simulink library "casper_library_delays"  (R2021a)
settings: Solver=ode45  StartTime=0.0  StopTime=10.0  RelTol=1e-3
libraries: xbsIndex_r4 x373, casper_library_misc x18, $bdroot x18, xbsReplacements_r4 x5, casper_library_multipliers x4, casper_library_downconverter x2
(part 1 of 5)
settings Model: Creator=mdexter  LastModifiedBy=jkocz
settings SolverCC: AlgebraicLoopSolver=TrustRegion
settings DataIOCC: LimitDataPoints=on  SaveFormat=Array  SignalLoggingSaveFormat=ModelDataLogs  ReturnWorkspaceOutputs=off
settings OptimizationCC: BlockReduction=off  BooleanDataType=off  ExpressionDepthLimit=2147483647  LifeSpan=inf
settings DebuggingCC: SaveWithParameterizedLinksMsg=none  UnderspecifiedInitializationDetection=Classic  MergeDetectMultiDrivingBlocksExec=none  SignalResolutionControl=TryResolveAllWithWarning  FcnCallInpInsideContextMsg=warning  AllowSymbolicDim=off  StateNameClashWarn=warning  SFUnexpectedBacktrackingDiag=warning  SFNoUnconditionalDefaultTransitionDiag=warning  SFExecutionAtInitializationDiag=none  SFMachineParentedDataDiag=warning  ArithmeticOperatorsInVariantConditions=warning
settings HardwareCC: ProdBitPerPointer=32  ProdBitPerSizeT=32  ProdBitPerPtrDiffT=32  ProdLargestAtomicFloat=None  ProdIntDivRoundTo=Undefined  ProdEndianess=Unspecified  ProdWordSize=32  ProdHWDeviceType=32-bit Generic  TargetUnknown=on
settings ModelReferenceCC: PropagateSignalLabelsOutOfModel=off
settings SFSimCC: SimUseLocalCustomCode=off  CustomCodeUndefinedFunction=UseInterfaceOnly
settings RTWCC: RTWUseLocalCustomCode=off
settings CodeAppCC: StateflowObjectComments=on
settings GRTTargetCC: TargetLangStandard=C89/C90 (ANSI)  CombineOutputUpdateFcns=off  GRTInterface=on
settings ConfigComp: CovMetricSettings=dw  CovSaveCumulativeToWorkspaceVar=on  CovSaveSingleToWorkspaceVar=on  CovExternalEMLEnable=off

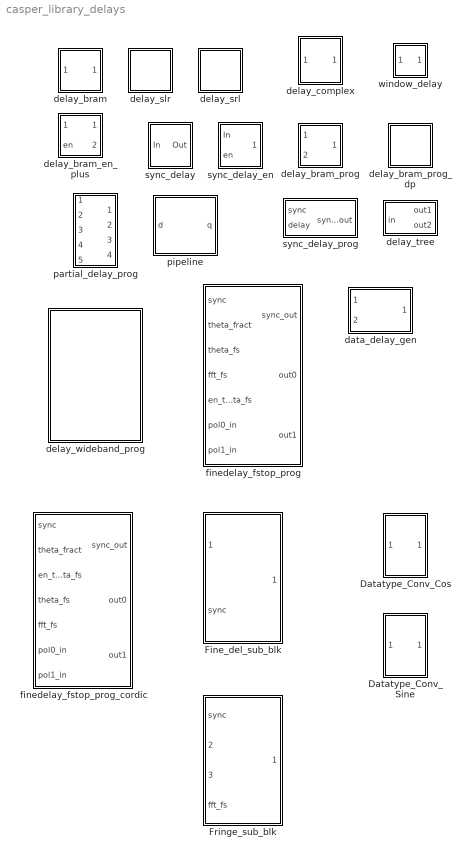
== system casper_library_delays ==
  Datatype_Conv_Cos : Subsystem  mask{theta_binary_bits=17, fft_bits=18}
      mask prompts: theta_binary_bits "Sine-Cos LUT Input binary point position"; fft_bits "FFT Input Bit Width"
  Datatype_Conv_Sine : Subsystem  mask{theta_binary_bits=17, fft_bits=18}
      mask prompts: theta_binary_bits "Sine-Cos LUT Input binary point position"; fft_bits "FFT Input Bit Width"
  Fine_del_sub_blk : Subsystem  mask{fft_len=1024, theta_bits=12, theta_binary_bits=9}
      mask prompts: fft_len "Number Of FFT Channels"; theta_bits "Sine-Cos LUT Input Bitwidth(Determines resolution of the phase)"; theta_binary_bits "Sine-Cos LUT Input binary point position"
      mask init:
      | low_limit = (2^theta_bits)*pi /8;
      | up_limit = (2^theta_bits)-((2^theta_bits)*pi /8);
  Fringe_sub_blk : Subsystem  mask{fft_len=1024, theta_bits=20, theta_binary_bits=17, fft_cycle_bits=17, sync_period=27}
      mask prompts: fft_len "Number Of FFT Channels"; theta_bits "Sine-Cos LUT Input Bitwidth (Determines the resolution of phase)"; theta_binary_bits "Sine-Cos LUT Input binary point position"; fft_cycle_bits "Maximum Number of FFT cycles  (Rate of change of Fringe ) = 2 ^ ?"; sync_period "Sync Period"
  data_delay_gen : Subsystem  mask(Delay_7){delaytype=sync_delay_prog, DelayLen=5, bram_latency=1, MaxDelay=1, use_dsp48=on}
      mask prompts: delaytype "delay type"; DelayLen "Delay by  [delay_bram, delay_slr, sync_delay, sync_delay_en, window_delay, pipeline]"; bram_latency "BRAM latency  [delay_bram]"; MaxDelay "Max Delay (2^?) [sync_delay_prog]"; use_dsp48 "Use DSP48 [delay_bram]"
      mask help: A combination of 7 different Delay blocks. Including delay_bram, delay_slr, sync_delay, sync_delay_en, sync_delay_prog, window_delay, pipeline.
      mask init:
      | config.source=str2func('delay_general');
      | config.name=delaytype;
      | config.toplevel=gcb;
      | xBlock(config, {delaytype, ...
      |                 {'Delaylen',DelayLen, ...
      |                 'MaxDelay', MaxDelay, ...
      |                 'use_dsp48', use_dsp48, ...
      |                 'bram_latency', bram_latency} }...
      |                 );
      settings: AttributesFormatString=Delay_7, %<delaytype>
      mask TypeOptions delaytype: delay_bram | delay_slr | sync_delay | sync_delay_en | sync_delay_prog | window_delay | pipeline
  delay_bram : Subsystem  mask(delay_bram){DelayLen=4, bram_latency=2, use_dsp48=off, async=off}
      mask prompts: DelayLen "Delay By:"; bram_latency "BRAM Latency"; use_dsp48 "Use DSP48"; async "asynchronous operation"
      mask help: A delay block that uses BRAM for its storage.
      mask init:
      | delay_bram_init(gcb, ...
      |     'DelayLen', DelayLen, ...
      |     'bram_latency', bram_latency, ...
      |     'use_dsp48', use_dsp48, ...
      |     'async', async);
      mask Help: eval('xlWeb(''http://casper.berkeley.edu/wiki/Delay_bram'')')
  delay_bram_en_plus : Subsystem  mask(delay_bram_en_plus){DelayLen=7, bram_latency=4}
      mask prompts: DelayLen "Enabled Delays:"; bram_latency "Extra (unenabled) delay for BRAM Latency"
      mask help:
      | A delay block that uses BRAM for its storage and only shifts when enabled.
      | However, BRAM latency cannot be enabled, so output appears <i>bram_latency</i>
      | clocks after an enable.
      mask init:
      | BitWidth = max(ceil(log2(DelayLen)), 2);
      mask Help: eval('xlWeb(''http://casper.berkeley.edu/wiki/Delay_bram_en_plus'')')
  delay_bram_prog : Subsystem  mask(delay_bram_prog){MaxDelay=7, bram_latency=4}
      mask prompts: MaxDelay "Max Delay (2^?):"; bram_latency "BRAM Latency"
      mask help:
      | A delay block that uses BRAM for its storage and has a run-time programmable
      | delay.  When delay is changed, some randomly determined samples will
      | be inserted/dropped from the buffered stream.
      mask Help: eval('xlWeb(''http://casper.berkeley.edu/wiki/Delay_bram_prog'')')
  delay_bram_prog_dp : Subsystem  mask(delay_bram_prog_dp){ram_bits=0, bram_latency=2, async=off}
      mask prompts: ram_bits "Max delay (2^?)"; bram_latency "BRAM latency"; async "asynchronous operation"
      mask init:
      | delay_bram_prog_dp_init(gcb, ...
      |     'ram_bits', ram_bits, ...
      |     'bram_latency', bram_latency, ...
      |     'async', async);
  delay_complex : Subsystem  mask(delay_complex){delay=6, n_bits=18, bin_pt=17, use_bram=1, bram_latency=3}
      mask prompts: delay "Delay Length"; n_bits "Sample Bit Width"; bin_pt "Binary Point"; use_bram "Use BRAM (0=no, 1=yes)"; bram_latency "BRAM Latency"
      mask help: A delay block that treats its input as complex, splits it into real and imaginary components, delays each component by a specified amount, and then re-joins them into a complex output. The underlying storage is user-selectable (either BRAM or SLR16 elements). The reason for this is wide (36 bit) delays make adjacent multipliers in multiplier-bram pairs unusable.
      mask init:
      | delay_complex_init(gcb, ...
      |     'delay', delay, ...
      |     'n_bits', n_bits, ...
      |     'bin_pt', bin_pt, ...
      |     'use_bram', use_bram, ...
      |     'bram_latency', bram_latency);
      settings: AttributesFormatString=|
      | depth = 6
      | delay_bram
      mask Help: eval('xlWeb(''http://casper.berkeley.edu/wiki/Delay_complex'')')
  delay_slr : Subsystem  mask(delay_slr){DelayLen=0, async=off}
      mask prompts: DelayLen "Delay by:"; async "asynchronous operation"
      mask help: A delay block that uses slices (SLR16s) for its storage.
      mask init:
      | delay_slr_init(gcb, ...
      |     'DelayLen', DelayLen, ...
      |     'async', async);
  delay_srl : Subsystem  mask(delay_srl){DelayLen=-1, async=off}
      mask prompts: DelayLen "Delay by:"; async "Asynchronous operation"
      mask help:
      | A delay block that uses slices (SRL16s) for its storage.
      |
      | It explicitly converts the first delay into a flip flop,
      | and lets XSG break up the remaining delays into a series
      | of SRL16+FF instances.
      |
      | This is advantageous because the setup time of an SRL is
      | longer than that of a flip flop.
      mask init:
      | delay_srl_init(gcb, ...
      |     'DelayLen', DelayLen, ...
      |     'async', async);
  delay_tree : Subsystem  mask(delay_tree){fanout=2, bfac=2}
      mask prompts: bfac "Branching factor"
      mask help: A tree of delays.
      mask init:
      | delay_tree_init(gcb, ...
      |     'fanout', fanout, ...
      |     'bfac', bfac);
      settings: AttributesFormatString=delay=2
  delay_wideband_prog : Subsystem  mask(delay_wideband_prog){max_delay=0, n_inputs_bits=2, bram_latency=2, bram_type=Dual Port, async=off}
      mask prompts: max_delay "Max Delay (Sample Clks)"; n_inputs_bits "Number of Simultaneous Inputs(2^?)"; bram_latency "BRAM Latency"; bram_type "Select type of BRAM"; async "asynchronous operation"
      mask init:
      | delay_wideband_prog_init(gcb,...
      |     'max_delay',max_delay,...
      |     'n_inputs_bits',n_inputs_bits,...
      |     'bram_latency',bram_latency,...
      |     'bram_type',bram_type, ...
      |     'async', async);
      mask TypeOptions bram_type: Single Port | Dual Port
  finedelay_fstop_prog : Subsystem  mask(finedelay_fstop_prog){n_input=2, fft_len=512, fft_bits=18, theta_bits=14, sine_cos_bits=18, fft_cycle_bits=12}
      mask prompts: n_input "Number of Simultaneous Inputs"; fft_len "Number Of FFT Channels"; fft_bits "FFT Input Bit Width"; theta_bits "Sine-Cos LUT Input Bitwidth (Determines the resolution of phase)"; sine_cos_bits "Sine-Cos LUT Output Data Width"; fft_cycle_bits "Maximum Number of FFT cycles  (Rate of change of Fringe ) = 2 ^ ?"
      mask init:
      | finedelay_fstop_prog_init(gcb,...
      |     'n_input',n_input,...
      |     'fft_len',fft_len,...
      |     'fft_bits',fft_bits,...
      |     'theta_bits',theta_bits,...
      |     'sine_cos_bits',sine_cos_bits,...
      |     'fft_cycle_bits',fft_cycle_bits);
  finedelay_fstop_prog_cordic : Subsystem  mask(finedelay_fstop_prog_cordic){n_input=2, fft_len=1024, fft_bits=18, theta_bits=20, theta_binary_bits=17, stages=9, fft_cycle_bits=17, sync_period=134217728}
      mask prompts: n_input "Number of Simultaneous Inputs"; fft_len "Number Of FFT Channels"; fft_bits "FFT Input Bit Width"; theta_bits "CORDIC Sine-Cos Input Bitwidth (Determines the resolution of phase)"; theta_binary_bits "CORDIC Sine-Cos Input Binary BitWidth"; stages "Number of Processing Elements of CORDIC block (integer value starting from 1)"; fft_cycle_bits "Maximum Number of FFT cycles  (Rate of change of Fringe ) = 2 ^ ?"; sync_period "Sync Period"
      mask init:
      | finedelay_fstop_prog_cordic_init(gcb,...
      |     'n_input',n_input,...
      |     'fft_len',fft_len,...
      |     'fft_bits',fft_bits,...
      |     'theta_bits',theta_bits,...
      |     'theta_binary_bits',theta_binary_bits,...
      |     'stages',stages,...
      |     'fft_cycle_bits',fft_cycle_bits,...
      |     'sync_period',sync_period);
  partial_delay_prog : Subsystem  mask(partial_delay){n_inputs=4, mux_latency=2}
      mask prompts: n_inputs "Number of Inputs (? >= 2)"; mux_latency "Mux Latency"
      mask help:
      | For a set of parallel inputs which represent consecutive time samples of the
      | same input signal, this block delays the stream by a dynamically selectable
      | number of samples between 0 and (n_inputs-1).
      mask init:
      | partial_delay_init(gcb, ...
      |     'n_inputs', n_inputs, ...
      |     'mux_latency', mux_latency);
      mask Help: eval('xlWeb(''http://casper.berkeley.edu/wiki/Partial_delay_prog'')')
  pipeline : Subsystem  mask(pipeline){csp_latency=3}
      mask prompts: csp_latency "Latency"
      mask help:
      | An explicitly laid-out delay line to avoid mapping to SRL16s
      | for use in pipelining to help achieve timing closure.
      mask init:
      | pipeline_init(gcb,'latency',csp_latency);
      settings: AttributesFormatString=Latency = %<latency>
      mask Display:
      | port_label('input', 1, 'd');
      | port_label('output', 1, 'q');
      | disp(['Z^-', num2str(csp_latency)]);
  sync_delay : Subsystem  mask(sync_delay){DelayLen=4}
      mask prompts: DelayLen "Delay Length:"
      mask help: Delay an infrequent boolean pulse by the specified number of clocks.
      mask init:
      | BitWidth = max(2, ceil(log2(DelayLen+1)));
      | UseCounter = 1;
      | if DelayLen == 0,
      | 	UseCounter = 0;
      | end
      mask Help: eval('xlWeb(''http://casper.berkeley.edu/wiki/Sync_delay'')')
      mask Display: fprintf('Z^-%d', DelayLen)
  sync_delay_en : Subsystem  mask(sync_delay_en){DelayLen=4}
      mask prompts: DelayLen "Delay Length:"
      mask help: Delay an infrequent boolean pulse by the specified number of enabled clocks.
      mask init:
      | BitWidth = max(2, ceil(log2(DelayLen+1)));
      | UseCounter = 1;
      | if DelayLen == 0,
      | 	UseCounter = 0;
      | end
      mask Help: eval('xlWeb(''http://casper.berkeley.edu/wiki/Sync_delay_en'')')
      mask Display:
      | fprintf('Z^-%d', DelayLen);
      | port_label('input',2,'en');
  sync_delay_prog : Subsystem  mask(sync_delay_prog){MaxDelay=4}
      mask prompts: MaxDelay "Max Delay (2^?):"
      mask help:
      | Delay an infrequent boolean pulse by  a run-time programmable number of enabled clocks.
      | If the input pulse repeats before the output pulse is generated, an internal counter
      | resets and that output pulse is never generated. When delay is changed, some randomly determined
      | samples will be inserted/dropped from the buffered stream.
      mask Help: eval('xlWeb(''http://casper.berkeley.edu/wiki/Sync_delay_prog'')')
  window_delay : Subsystem  mask{delay=10}
      mask prompts: delay "desired delay (>2)"
      mask Display: fprintf('Z^-%d', delay)

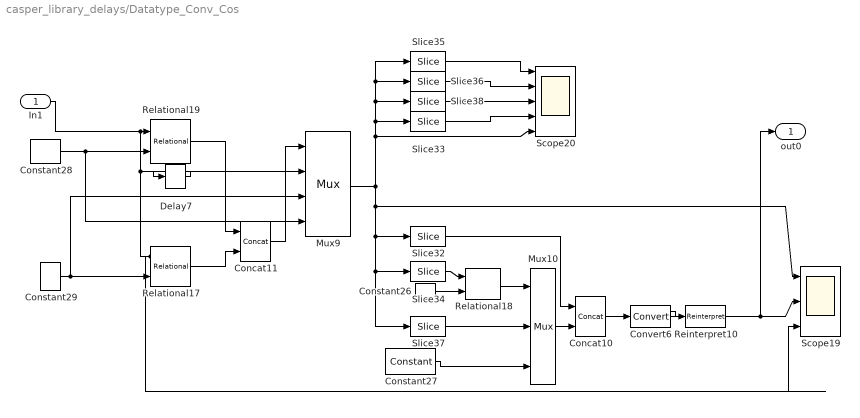
== system casper_library_delays/Datatype_Conv_Cos ==
  In1 : Inport
  Concat10 : xbsIndex_r4/Concat  num_inputs=2  dbl_ovrd=off  block_type=concat
      settings: block_version=10.1.3
  Concat11 : xbsIndex_r4/Concat  num_inputs=2  dbl_ovrd=off  block_type=concat
      settings: block_version=10.1.3
  Constant26 : xbsIndex_r4/Constant  const=1  gui_display_data_type=Fixed-point  arith_type=Unsigned  n_bits=3  bin_pt=0  preci_type=Single  exp_width=8  frac_width=24  explicit_period=off  period=1  equ=P=C  opselect=C  inp2=PCIN>>17  opr=+  inp1=P  carry=CIN  dbl_ovrd=off  block_type=constant
  Constant27 : xbsIndex_r4/Constant  const=2^(theta_binary_bits)-1  gui_display_data_type=Fixed-point  arith_type=Unsigned  n_bits=theta_binary_bits  bin_pt=0  preci_type=Single  exp_width=8  frac_width=24  explicit_period=off  period=1  equ=P=C  opselect=C  inp2=PCIN>>17  opr=+  inp1=P  carry=CIN  dbl_ovrd=off  block_type=constant
  Constant28 : xbsIndex_r4/Constant  const=1  gui_display_data_type=Fixed-point  arith_type=Signed (2's comp)  n_bits=20  bin_pt=17  preci_type=Single  exp_width=8  frac_width=24  explicit_period=off  period=1  equ=P=C  opselect=C  inp2=PCIN>>17  opr=+  inp1=P  carry=CIN  dbl_ovrd=off  block_type=constant
  Constant29 : xbsIndex_r4/Constant  const=-1  gui_display_data_type=Fixed-point  arith_type=Signed (2's comp)  n_bits=20  bin_pt=17  preci_type=Single  exp_width=8  frac_width=24  explicit_period=off  period=1  equ=P=C  opselect=C  inp2=PCIN>>17  opr=+  inp1=P  carry=CIN  dbl_ovrd=off  block_type=constant
  Convert6 : xbsIndex_r4/Convert  gui_display_data_type=Fixed-point  arith_type="Signed  (2's comp)"  n_bits=fft_bits  bin_pt=0  float_type=Single  exp_bits=8  fraction_bits=24  quantization=Truncate  overflow=Wrap  en=off  latency=0  pipeline=off  dbl_ovrd=off  block_type=convert
      settings: block_version=10.1.3
  Delay7 : xbsIndex_r4/Delay  rst=off  infoeditControl=Selection of Reset will increase slice count due to use of real FFs and instead of SRLs  en=off  latency=1  reg_retiming=off  dbl_ovrd=off  block_type=delay
  Mux10 : xbsIndex_r4/Mux  inputs=2  en=off  latency=0  precision=Full  arith_type=Unsigned  n_bits=16  bin_pt=14  quantization=Truncate  overflow=Wrap  dbl_ovrd=off  block_type=mux
  Mux9 : xbsIndex_r4/Mux  inputs=3  en=off  latency=0  precision=Full  arith_type=Unsigned  n_bits=16  bin_pt=14  quantization=Truncate  overflow=Wrap  dbl_ovrd=off  block_type=mux
  Reinterpret10 : xbsIndex_r4/Reinterpret  force_arith_type=off  arith_type=Unsigned  force_bin_pt=on  bin_pt=fft_bits-1  block_type=reinterpret
      settings: infoedit="Changes signal type without altering the binary representation.   You can changed the signal between signed and unsigned, and relocate the binary point.<P><P>Hardware notes: In hardware this block costs nothing.<P><P>Example:  Suppose the input is 6 bits wide, signed, with 2 fractional bits, and the output is forced to unsigned with 0 fractional bits.  Then an input of -2.0 (1110.00 in binary 2's complement) becomes an output of 56 (111000 in binary)."  block_version=10.1.3
  Relational17 : xbsIndex_r4/Relational  mode=a<b  op_type=Bool  en=off  latency=1  dbl_ovrd=off  block_type=relational
      settings: block_version=10.1.3
  Relational18 : xbsIndex_r4/Relational  mode=a=b  op_type=Bool  en=off  latency=0  dbl_ovrd=off  block_type=relational
      settings: block_version=10.1.3
  Relational19 : xbsIndex_r4/Relational  mode=a>b  op_type=Bool  en=off  latency=1  dbl_ovrd=off  block_type=relational
      settings: block_version=10.1.3
  Scope19 : Scope  NumInputPorts=3
  Scope20 : Scope  NumInputPorts=5
  Slice32 : xbsIndex_r4/Slice  nbits=1  boolean_output=off  mode=Upper Bit Location + Width  bit1=0  base1=MSB of Input  bit0=0  base0=LSB of Input  dbl_ovrd=off  block_type=slice
      settings: infoedit="Extracts a given range of bits from each input sample and presents it at the output.  The output type is ordinarily unsigned with binary point at zero, but can be Boolean when the slice is one bit wide.<P><P>Hardware notes: In hardware this block costs nothing."  block_version=10.1.3
  Slice33 : xbsIndex_r4/Slice  nbits=3  boolean_output=off  mode=Upper Bit Location + Width  bit1=0  base1=MSB of Input  bit0=0  base0=LSB of Input  dbl_ovrd=off  block_type=slice
      settings: infoedit="Extracts a given range of bits from each input sample and presents it at the output.  The output type is ordinarily unsigned with binary point at zero, but can be Boolean when the slice is one bit wide.<P><P>Hardware notes: In hardware this block costs nothing."  block_version=10.1.3
  Slice34 : xbsIndex_r4/Slice  nbits=3  boolean_output=off  mode=Upper Bit Location + Width  bit1=0  base1=MSB of Input  bit0=0  base0=LSB of Input  dbl_ovrd=off  block_type=slice
      settings: infoedit="Extracts a given range of bits from each input sample and presents it at the output.  The output type is ordinarily unsigned with binary point at zero, but can be Boolean when the slice is one bit wide.<P><P>Hardware notes: In hardware this block costs nothing."  block_version=10.1.3
  Slice35 : xbsIndex_r4/Slice  nbits=1  boolean_output=off  mode=Upper Bit Location + Width  bit1=0  base1=MSB of Input  bit0=0  base0=LSB of Input  dbl_ovrd=off  block_type=slice
      settings: infoedit="Extracts a given range of bits from each input sample and presents it at the output.  The output type is ordinarily unsigned with binary point at zero, but can be Boolean when the slice is one bit wide.<P><P>Hardware notes: In hardware this block costs nothing."  block_version=10.1.3
  Slice36 : xbsIndex_r4/Slice  nbits=1  boolean_output=off  mode=Upper Bit Location + Width  bit1=-1  base1=MSB of Input  bit0=0  base0=LSB of Input  dbl_ovrd=off  block_type=slice
      settings: infoedit="Extracts a given range of bits from each input sample and presents it at the output.  The output type is ordinarily unsigned with binary point at zero, but can be Boolean when the slice is one bit wide.<P><P>Hardware notes: In hardware this block costs nothing."  block_version=10.1.3
  Slice37 : xbsIndex_r4/Slice  nbits=theta_binary_bits  boolean_output=off  mode=Lower Bit Location + Width  bit1=0  base1=MSB of Input  bit0=0  base0=LSB of Input  dbl_ovrd=off  block_type=slice
      settings: infoedit="Extracts a given range of bits from each input sample and presents it at the output.  The output type is ordinarily unsigned with binary point at zero, but can be Boolean when the slice is one bit wide.<P><P>Hardware notes: In hardware this block costs nothing."  block_version=10.1.3
  Slice38 : xbsIndex_r4/Slice  nbits=1  boolean_output=off  mode=Upper Bit Location + Width  bit1=-2  base1=MSB of Input  bit0=0  base0=LSB of Input  dbl_ovrd=off  block_type=slice
      settings: infoedit="Extracts a given range of bits from each input sample and presents it at the output.  The output type is ordinarily unsigned with binary point at zero, but can be Boolean when the slice is one bit wide.<P><P>Hardware notes: In hardware this block costs nothing."  block_version=10.1.3
  out0 : Outport  VectorParamsAs1DForOutWhenUnconnected=off
  wires:
  In1/1 -> Relational19/1, Delay7/1, Relational17/1, Scope19/3
  Slice33/1 -> Scope20/4
  Slice38/1 -> Scope20/3
  Slice36/1 -> Scope20/2
  Slice35/1 -> Scope20/1
  Reinterpret10/1 -> Scope19/2, out0/1
  Convert6/1 -> Reinterpret10/1
  Concat10/1 -> Convert6/1
  Constant27/1 -> Mux10/3
  Slice37/1 -> Mux10/2
  Mux10/1 -> Concat10/2
  Relational18/1 -> Mux10/1
  Constant26/1 -> Relational18/2
  Slice34/1 -> Relational18/1
  Slice32/1 -> Concat10/1
  Mux9/1 -> Slice32/1, Slice34/1, Slice37/1, Scope19/1, Slice36/1, Slice35/1, Slice38/1, Slice33/1, Scope20/5
  Constant28/1 -> Relational19/2, Mux9/4
  Delay7/1 -> Mux9/2
  Concat11/1 -> Mux9/1
  Relational19/1 -> Concat11/1
  Relational17/1 -> Concat11/2
  Constant29/1 -> Relational17/2, Mux9/3

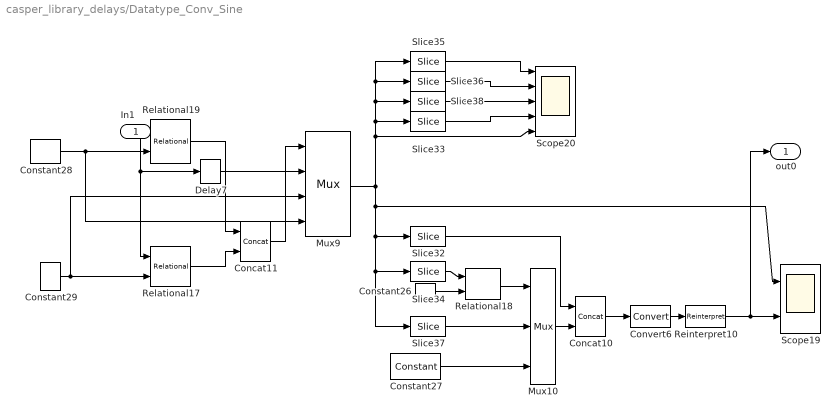
== system casper_library_delays/Datatype_Conv_Sine ==
  In1 : Inport
  Concat10 : xbsIndex_r4/Concat  num_inputs=2  dbl_ovrd=off  block_type=concat
      settings: block_version=10.1.3
  Concat11 : xbsIndex_r4/Concat  num_inputs=2  dbl_ovrd=off  block_type=concat
      settings: block_version=10.1.3
  Constant26 : xbsIndex_r4/Constant  const=1  gui_display_data_type=Fixed-point  arith_type=Unsigned  n_bits=3  bin_pt=0  preci_type=Single  exp_width=8  frac_width=24  explicit_period=off  period=1  equ=P=C  opselect=C  inp2=PCIN>>17  opr=+  inp1=P  carry=CIN  dbl_ovrd=off  block_type=constant
  Constant27 : xbsIndex_r4/Constant  const=2^(theta_binary_bits)-1  gui_display_data_type=Fixed-point  arith_type=Unsigned  n_bits=theta_binary_bits  bin_pt=0  preci_type=Single  exp_width=8  frac_width=24  explicit_period=off  period=1  equ=P=C  opselect=C  inp2=PCIN>>17  opr=+  inp1=P  carry=CIN  dbl_ovrd=off  block_type=constant
  Constant28 : xbsIndex_r4/Constant  const=1  gui_display_data_type=Fixed-point  arith_type=Signed (2's comp)  n_bits=20  bin_pt=17  preci_type=Single  exp_width=8  frac_width=24  explicit_period=off  period=1  equ=P=C  opselect=C  inp2=PCIN>>17  opr=+  inp1=P  carry=CIN  dbl_ovrd=off  block_type=constant
  Constant29 : xbsIndex_r4/Constant  const=-1  gui_display_data_type=Fixed-point  arith_type=Signed (2's comp)  n_bits=20  bin_pt=17  preci_type=Single  exp_width=8  frac_width=24  explicit_period=off  period=1  equ=P=C  opselect=C  inp2=PCIN>>17  opr=+  inp1=P  carry=CIN  dbl_ovrd=off  block_type=constant
  Convert6 : xbsIndex_r4/Convert  gui_display_data_type=Fixed-point  arith_type="Signed  (2's comp)"  n_bits=fft_bits  bin_pt=0  float_type=Single  exp_bits=8  fraction_bits=24  quantization=Truncate  overflow=Wrap  en=off  latency=0  pipeline=off  dbl_ovrd=off  block_type=convert
      settings: block_version=10.1.3
  Delay7 : xbsIndex_r4/Delay  rst=off  infoeditControl=Selection of Reset will increase slice count due to use of real FFs and instead of SRLs  en=off  latency=1  reg_retiming=off  dbl_ovrd=off  block_type=delay
  Mux10 : xbsIndex_r4/Mux  inputs=2  en=off  latency=0  precision=Full  arith_type=Unsigned  n_bits=16  bin_pt=14  quantization=Truncate  overflow=Wrap  dbl_ovrd=off  block_type=mux
  Mux9 : xbsIndex_r4/Mux  inputs=3  en=off  latency=0  precision=Full  arith_type=Unsigned  n_bits=16  bin_pt=14  quantization=Truncate  overflow=Wrap  dbl_ovrd=off  block_type=mux
  Reinterpret10 : xbsIndex_r4/Reinterpret  force_arith_type=off  arith_type=Unsigned  force_bin_pt=on  bin_pt=fft_bits-1  block_type=reinterpret
      settings: infoedit="Changes signal type without altering the binary representation.   You can changed the signal between signed and unsigned, and relocate the binary point.<P><P>Hardware notes: In hardware this block costs nothing.<P><P>Example:  Suppose the input is 6 bits wide, signed, with 2 fractional bits, and the output is forced to unsigned with 0 fractional bits.  Then an input of -2.0 (1110.00 in binary 2's complement) becomes an output of 56 (111000 in binary)."  block_version=10.1.3
  Relational17 : xbsIndex_r4/Relational  mode=a<b  op_type=Bool  en=off  latency=1  dbl_ovrd=off  block_type=relational
      settings: block_version=10.1.3
  Relational18 : xbsIndex_r4/Relational  mode=a=b  op_type=Bool  en=off  latency=0  dbl_ovrd=off  block_type=relational
      settings: block_version=10.1.3
  Relational19 : xbsIndex_r4/Relational  mode=a>b  op_type=Bool  en=off  latency=1  dbl_ovrd=off  block_type=relational
      settings: block_version=10.1.3
  Scope19 : Scope  NumInputPorts=2
  Scope20 : Scope  NumInputPorts=5
  Slice32 : xbsIndex_r4/Slice  nbits=1  boolean_output=off  mode=Upper Bit Location + Width  bit1=0  base1=MSB of Input  bit0=0  base0=LSB of Input  dbl_ovrd=off  block_type=slice
      settings: infoedit="Extracts a given range of bits from each input sample and presents it at the output.  The output type is ordinarily unsigned with binary point at zero, but can be Boolean when the slice is one bit wide.<P><P>Hardware notes: In hardware this block costs nothing."  block_version=10.1.3
  Slice33 : xbsIndex_r4/Slice  nbits=3  boolean_output=off  mode=Upper Bit Location + Width  bit1=0  base1=MSB of Input  bit0=0  base0=LSB of Input  dbl_ovrd=off  block_type=slice
      settings: infoedit="Extracts a given range of bits from each input sample and presents it at the output.  The output type is ordinarily unsigned with binary point at zero, but can be Boolean when the slice is one bit wide.<P><P>Hardware notes: In hardware this block costs nothing."  block_version=10.1.3
  Slice34 : xbsIndex_r4/Slice  nbits=3  boolean_output=off  mode=Upper Bit Location + Width  bit1=0  base1=MSB of Input  bit0=0  base0=LSB of Input  dbl_ovrd=off  block_type=slice
      settings: infoedit="Extracts a given range of bits from each input sample and presents it at the output.  The output type is ordinarily unsigned with binary point at zero, but can be Boolean when the slice is one bit wide.<P><P>Hardware notes: In hardware this block costs nothing."  block_version=10.1.3
  Slice35 : xbsIndex_r4/Slice  nbits=1  boolean_output=off  mode=Upper Bit Location + Width  bit1=0  base1=MSB of Input  bit0=0  base0=LSB of Input  dbl_ovrd=off  block_type=slice
      settings: infoedit="Extracts a given range of bits from each input sample and presents it at the output.  The output type is ordinarily unsigned with binary point at zero, but can be Boolean when the slice is one bit wide.<P><P>Hardware notes: In hardware this block costs nothing."  block_version=10.1.3
  Slice36 : xbsIndex_r4/Slice  nbits=1  boolean_output=off  mode=Upper Bit Location + Width  bit1=-1  base1=MSB of Input  bit0=0  base0=LSB of Input  dbl_ovrd=off  block_type=slice
      settings: infoedit="Extracts a given range of bits from each input sample and presents it at the output.  The output type is ordinarily unsigned with binary point at zero, but can be Boolean when the slice is one bit wide.<P><P>Hardware notes: In hardware this block costs nothing."  block_version=10.1.3
  Slice37 : xbsIndex_r4/Slice  nbits=theta_binary_bits  boolean_output=off  mode=Lower Bit Location + Width  bit1=0  base1=MSB of Input  bit0=0  base0=LSB of Input  dbl_ovrd=off  block_type=slice
      settings: infoedit="Extracts a given range of bits from each input sample and presents it at the output.  The output type is ordinarily unsigned with binary point at zero, but can be Boolean when the slice is one bit wide.<P><P>Hardware notes: In hardware this block costs nothing."  block_version=10.1.3
  Slice38 : xbsIndex_r4/Slice  nbits=1  boolean_output=off  mode=Upper Bit Location + Width  bit1=-2  base1=MSB of Input  bit0=0  base0=LSB of Input  dbl_ovrd=off  block_type=slice
      settings: infoedit="Extracts a given range of bits from each input sample and presents it at the output.  The output type is ordinarily unsigned with binary point at zero, but can be Boolean when the slice is one bit wide.<P><P>Hardware notes: In hardware this block costs nothing."  block_version=10.1.3
  out0 : Outport  VectorParamsAs1DForOutWhenUnconnected=off
  wires:
  Constant29/1 -> Mux9/3, Relational17/2
  Relational17/1 -> Concat11/2
  Relational19/1 -> Concat11/1
  Concat11/1 -> Mux9/1
  Delay7/1 -> Mux9/2
  Constant28/1 -> Mux9/4, Relational19/2
  Mux9/1 -> Scope20/5, Slice33/1, Slice38/1, Slice35/1, Slice36/1, Scope19/1, Slice37/1, Slice34/1, Slice32/1
  Slice32/1 -> Concat10/1
  Slice34/1 -> Relational18/1
  Constant26/1 -> Relational18/2
  Relational18/1 -> Mux10/1
  Mux10/1 -> Concat10/2
  Slice37/1 -> Mux10/2
  Constant27/1 -> Mux10/3
  Concat10/1 -> Convert6/1
  Convert6/1 -> Reinterpret10/1
  Reinterpret10/1 -> Scope19/2, out0/1
  Slice35/1 -> Scope20/1
  Slice36/1 -> Scope20/2
  Slice38/1 -> Scope20/3
  Slice33/1 -> Scope20/4
  In1/1 -> Delay7/1, Relational17/1, Relational19/1

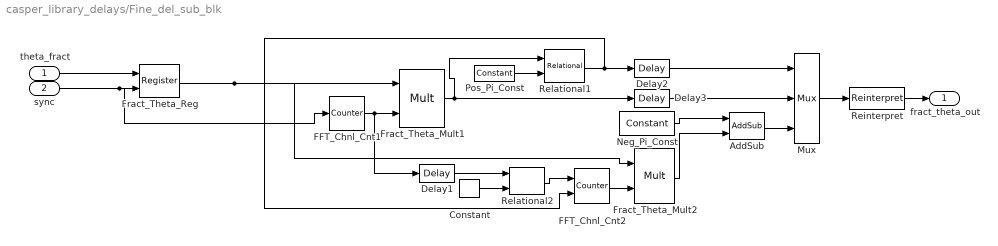
== system casper_library_delays/Fine_del_sub_blk ==
  theta_fract : Inport
  sync : Inport  Port=2
  AddSub : xbsIndex_r4/AddSub  mode=Addition  use_carryin=off  use_carryout=off  en=off  latency=0  precision=User Defined  arith_type=Unsigned  n_bits=theta_bits  bin_pt=0  quantization=Truncate  overflow=Wrap  use_behavioral_HDL=off  hw_selection=Fabric  pipelined=off  use_rpm=on  dbl_ovrd=off  block_type=addsub
      settings: block_version=10.1.3
  Constant : xbsIndex_r4/Constant  const=0  gui_display_data_type=Fixed-point  arith_type=Unsigned  n_bits=10  bin_pt=0  preci_type=Single  exp_width=8  frac_width=24  explicit_period=off  period=1  equ=P=C  opselect=C  inp2=PCIN>>17  opr=+  inp1=P  carry=CIN  dbl_ovrd=off  block_type=constant
  Delay1 : xbsIndex_r4/Delay  rst=off  infoeditControl=Selection of Reset will increase slice count due to use of real FFs and instead of SRLs  en=off  latency=3  reg_retiming=off  dbl_ovrd=off  block_type=delay
  Delay2 : xbsIndex_r4/Delay  rst=off  infoeditControl=Selection of Reset will increase slice count due to use of real FFs and instead of SRLs  en=off  latency=3  reg_retiming=off  dbl_ovrd=off  block_type=delay
  Delay3 : xbsIndex_r4/Delay  rst=off  infoeditControl=Selection of Reset will increase slice count due to use of real FFs and instead of SRLs  en=off  latency=3  reg_retiming=off  dbl_ovrd=off  block_type=delay
  FFT_Chnl_Cnt1 : xbsIndex_r4/Counter  cnt_type=Free Running  cnt_to=Inf  operation=Up  start_count=0  cnt_by_val=2  arith_type=Unsigned  n_bits=ceil(log2(fft_len))  bin_pt=0  load_pin=off  rst=on  en=off  explicit_period=on  period=1  use_behavioral_HDL=off  implementation=Fabric  use_rpm=on  dbl_ovrd=off  block_type=counter
      settings: xl_area=[0, 0, 0, 0, 0, 0, 0]
  FFT_Chnl_Cnt2 : xbsIndex_r4/Counter  cnt_type=Free Running  cnt_to=Inf  operation=Up  start_count=0  cnt_by_val=2  arith_type=Unsigned  n_bits=ceil(log2(fft_len))  bin_pt=0  load_pin=off  rst=on  en=on  explicit_period=on  period=1  use_behavioral_HDL=off  implementation=Fabric  use_rpm=on  dbl_ovrd=off  block_type=counter
      settings: xl_area=[0, 0, 0, 0, 0, 0, 0]
  Fract_Theta_Mult1 : xbsIndex_r4/Mult  precision=User Defined  arith_type=Unsigned  n_bits=theta_bits  bin_pt=0  quantization=Truncate  overflow=Wrap  en=off  latency=3  use_behavioral_HDL=off  opt=Speed  use_embedded=on  optimum_pipeline=off  pipeline=on  dbl_ovrd=off  use_rpm=on  placement_style=Rectangular shape  block_type=mult
      settings: infoedit=Hardware notes: To use the internal pipeline stage of the dedicated multiplier you must select 'Pipeline for maximum performance'.  xl_area=[0, 0, 0, 0, 0, 0, 0]  block_version=10.1.3
  Fract_Theta_Mult2 : xbsIndex_r4/Mult  precision=User Defined  arith_type=Unsigned  n_bits=theta_bits  bin_pt=0  quantization=Truncate  overflow=Wrap  en=off  latency=3  use_behavioral_HDL=off  opt=Speed  use_embedded=on  optimum_pipeline=off  pipeline=on  dbl_ovrd=off  use_rpm=on  placement_style=Rectangular shape  block_type=mult
      settings: infoedit=Hardware notes: To use the internal pipeline stage of the dedicated multiplier you must select 'Pipeline for maximum performance'.  xl_area=[0, 0, 0, 0, 0, 0, 0]  block_version=10.1.3
  Fract_Theta_Reg : xbsIndex_r4/Register  init=0  rst=off  en=on  dbl_ovrd=off  block_type=register
      settings: xl_area=[0, 0, 0, 0, 0, 0, 0]
  Mux : xbsIndex_r4/Mux  inputs=2  en=off  latency=0  precision=Full  arith_type=Unsigned  n_bits=16  bin_pt=14  quantization=Truncate  overflow=Wrap  dbl_ovrd=off  block_type=mux
  Neg_Pi_Const : xbsIndex_r4/Constant  const=up_limit  gui_display_data_type=Fixed-point  arith_type=Unsigned  n_bits=theta_bits  bin_pt=0  preci_type=Single  exp_width=8  frac_width=24  explicit_period=off  period=1  equ=P=C  opselect=C  inp2=PCIN>>17  opr=+  inp1=P  carry=CIN  dbl_ovrd=off  block_type=constant
  Pos_Pi_Const : xbsIndex_r4/Constant  const=low_limit  gui_display_data_type=Fixed-point  arith_type=Unsigned  n_bits=theta_bits  bin_pt=0  preci_type=Single  exp_width=8  frac_width=24  explicit_period=off  period=1  equ=P=C  opselect=C  inp2=PCIN>>17  opr=+  inp1=P  carry=CIN  dbl_ovrd=off  block_type=constant
  Reinterpret : xbsIndex_r4/Reinterpret  force_arith_type=on  arith_type="Signed  (2's comp)"  force_bin_pt=on  bin_pt=theta_binary_bits  block_type=reinterpret
      settings: infoedit="Changes signal type without altering the binary representation.   You can changed the signal between signed and unsigned, and relocate the binary point.<P><P>Hardware notes: In hardware this block costs nothing.<P><P>Example:  Suppose the input is 6 bits wide, signed, with 2 fractional bits, and the output is forced to unsigned with 0 fractional bits.  Then an input of -2.0 (1110.00 in binary 2's complement) becomes an output of 56 (111000 in binary)."  block_version=10.1.3
  Relational1 : xbsIndex_r4/Relational  mode=a>=b  op_type=Bool  en=off  latency=0  dbl_ovrd=off  block_type=relational
      settings: block_version=10.1.3
  Relational2 : xbsIndex_r4/Relational  mode=a=b  op_type=Bool  en=off  latency=0  dbl_ovrd=off  block_type=relational
      settings: block_version=10.1.3
  fract_theta_out : Outport  VectorParamsAs1DForOutWhenUnconnected=off
  wires:
  Relational2/1 -> FFT_Chnl_Cnt2/1
  Delay1/1 -> Relational2/1
  Reinterpret/1 -> fract_theta_out/1
  sync/1 -> FFT_Chnl_Cnt1/1, Fract_Theta_Reg/2
  theta_fract/1 -> Fract_Theta_Reg/1
  Delay2/1 -> Mux/1
  FFT_Chnl_Cnt2/1 -> Fract_Theta_Mult2/2
  Delay3/1 -> Mux/2
  Constant/1 -> Relational2/2
  Fract_Theta_Mult2/1 -> AddSub/2
  Mux/1 -> Reinterpret/1
  AddSub/1 -> Mux/3
  Neg_Pi_Const/1 -> AddSub/1
  Relational1/1 -> FFT_Chnl_Cnt2/2, Delay2/1
  Pos_Pi_Const/1 -> Relational1/2
  Fract_Theta_Mult1/1 -> Relational1/1, Delay3/1
  FFT_Chnl_Cnt1/1 -> Delay1/1, Fract_Theta_Mult1/2
  Fract_Theta_Reg/1 -> Fract_Theta_Mult2/1, Fract_Theta_Mult1/1

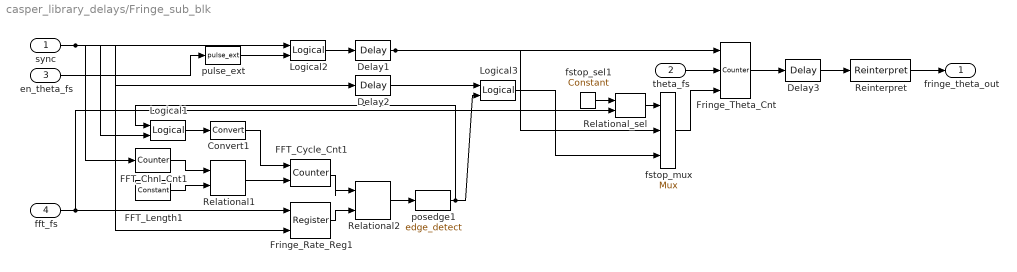
== system casper_library_delays/Fringe_sub_blk ==
  sync : Inport
  theta_fs : Inport  Port=2
  en_theta_fs : Inport  Port=3
  fft_fs : Inport  Port=4
  Convert1 : xbsIndex_r4/Convert  gui_display_data_type=Fixed-point  arith_type=Boolean  n_bits=8  bin_pt=6  float_type=Single  exp_bits=8  fraction_bits=24  quantization=Truncate  overflow=Wrap  en=off  latency=0  pipeline=off  dbl_ovrd=off  block_type=convert
      settings: xl_area=[0, 0, 0, 0, 0, 0, 0]  block_version=10.1.3
  Delay1 : xbsIndex_r4/Delay  rst=off  infoeditControl=Selection of Reset will increase slice count due to use of real FFs and instead of SRLs  en=off  latency=1  reg_retiming=off  dbl_ovrd=off  block_type=delay
      settings: xl_area=[0, 0, 0, 0, 0, 0, 0]
  Delay2 : xbsIndex_r4/Delay  rst=off  infoeditControl=Selection of Reset will increase slice count due to use of real FFs and instead of SRLs  en=off  latency=1  reg_retiming=off  dbl_ovrd=off  block_type=delay
      settings: xl_area=[0, 0, 0, 0, 0, 0, 0]
  Delay3 : xbsIndex_r4/Delay  rst=off  infoeditControl=Selection of Reset will increase slice count due to use of real FFs and instead of SRLs  en=off  latency=2  reg_retiming=off  dbl_ovrd=off  block_type=delay
      settings: xl_area=[0, 0, 0, 0, 0, 0, 0]
  FFT_Chnl_Cnt1 : xbsIndex_r4/Counter  cnt_type=Free Running  cnt_to=Inf  operation=Up  start_count=0  cnt_by_val=1  arith_type=Unsigned  n_bits=(ceil(log2(fft_len)))-1  bin_pt=0  load_pin=off  rst=on  en=off  explicit_period=off  period=1  use_behavioral_HDL=off  implementation=Fabric  use_rpm=on  dbl_ovrd=off  block_type=counter
      settings: xl_area=[0, 0, 0, 0, 0, 0, 0]
  FFT_Cycle_Cnt1 : xbsIndex_r4/Counter  cnt_type=Free Running  cnt_to=Inf  operation=Up  start_count=0  cnt_by_val=1  arith_type=Unsigned  n_bits=fft_cycle_bits  bin_pt=0  load_pin=off  rst=on  en=on  explicit_period=off  period=1  use_behavioral_HDL=off  implementation=Fabric  use_rpm=on  dbl_ovrd=off  block_type=counter
      settings: xl_area=[0, 0, 0, 0, 0, 0, 0]
  FFT_Length1 : xbsIndex_r4/Constant  const=(fft_len/2)-1  gui_display_data_type=Fixed-point  arith_type=Unsigned  n_bits=(ceil(log2(fft_len))) -1  bin_pt=0  preci_type=Single  exp_width=8  frac_width=24  explicit_period=on  period=1  equ=P=C  opselect=C  inp2=PCIN>>17  opr=+  inp1=P  carry=CIN  dbl_ovrd=off  block_type=constant
  Fringe_Rate_Reg1 : xbsIndex_r4/Register  init=0  rst=off  en=on  dbl_ovrd=off  block_type=register
      settings: xl_area=[0, 0, 0, 0, 0, 0, 0]
  Fringe_Theta_Cnt : xbsIndex_r4/Counter  cnt_type=Free Running  cnt_to=Inf  operation=Up  start_count=0  cnt_by_val=1  arith_type=Unsigned  n_bits=theta_bits  bin_pt=0  load_pin=on  rst=off  en=on  explicit_period=on  period=1  use_behavioral_HDL=off  implementation=Fabric  use_rpm=on  dbl_ovrd=off  block_type=counter
      settings: xl_area=[0, 0, 0, 0, 0, 0, 0]
  Logical1 : xbsIndex_r4/Logical  logical_function=OR  inputs=2  en=off  latency=0  precision=Full  arith_type=Unsigned  n_bits=1  bin_pt=0  align_bp=on  dbl_ovrd=off  block_type=logical
      settings: xl_area=[0, 0, 0, 0, 0, 0, 0]
  Logical2 : xbsIndex_r4/Logical  logical_function=AND  inputs=2  en=off  latency=0  precision=Full  arith_type=Unsigned  n_bits=1  bin_pt=0  align_bp=on  dbl_ovrd=off  block_type=logical
      settings: xl_area=[0, 0, 0, 0, 0, 0, 0]
  Logical3 : xbsIndex_r4/Logical  logical_function=OR  inputs=2  en=off  latency=0  precision=Full  arith_type=Unsigned  n_bits=1  bin_pt=0  align_bp=on  dbl_ovrd=off  block_type=logical
      settings: xl_area=[0, 0, 0, 0, 0, 0, 0]
  Reinterpret : xbsIndex_r4/Reinterpret  force_arith_type=on  arith_type="Signed  (2's comp)"  force_bin_pt=on  bin_pt=theta_binary_bits  block_type=reinterpret
      settings: infoedit="Changes signal type without altering the binary representation.   You can changed the signal between signed and unsigned, and relocate the binary point.<P><P>Hardware notes: In hardware this block costs nothing.<P><P>Example:  Suppose the input is 6 bits wide, signed, with 2 fractional bits, and the output is forced to unsigned with 0 fractional bits.  Then an input of -2.0 (1110.00 in binary 2's complement) becomes an output of 56 (111000 in binary)."  block_version=10.1.3
  Relational1 : xbsIndex_r4/Relational  mode=a=b  op_type=Bool  en=off  latency=0  dbl_ovrd=off  block_type=relational
      settings: xl_area=[0, 0, 0, 0, 0, 0, 0]  block_version=10.1.3
  Relational2 : xbsIndex_r4/Relational  mode=a=b  op_type=Bool  en=off  latency=0  dbl_ovrd=off  block_type=relational
      settings: xl_area=[0, 0, 0, 0, 0, 0, 0]  block_version=10.1.3
  Relational_sel : xbsIndex_r4/Relational  mode=a!=b  op_type=Bool  en=off  latency=0  dbl_ovrd=off  block_type=relational
      settings: xl_area=[0, 0, 0, 0, 0, 0, 0]  block_version=10.1.3
  fstop_mux : xbsIndex_r4/Mux  inputs=2  en=off  latency=0  precision=Full  arith_type="Signed  (2's comp)"  n_bits=8  bin_pt=2  quantization=Truncate  overflow=Wrap  dbl_ovrd=off  block_type=mux
      settings: xl_area=[0, 0, 0, 0, 0, 0, 0]
  fstop_sel1 : xbsIndex_r4/Constant  const=0  gui_display_data_type=Fixed-point  arith_type=Unsigned  n_bits=17  bin_pt=0  preci_type=Single  exp_width=8  frac_width=24  explicit_period=on  period=1  equ=P=C  opselect=C  inp2=PCIN>>17  opr=+  inp1=P  carry=CIN  dbl_ovrd=off  block_type=constant
  posedge1 : casper_library_misc/edge_detect  edge=Rising  polarity=Active High  x_in=[0 0.08 0.08 0.16 0.16 0.24 0.24 0.32 0.32 0.4]  y_in="[-1 -1  1  1  1  1  1  1  1  1]"  x_out=[0.6 0.68 0.68 0.76 0.76 0.84 0.84 0.92 0.92 1]  y_out="[-1 -1  1  1 -1 -1 -1 -1 -1 -1]"
  pulse_ext : casper_library_misc/pulse_ext  pulse_len=sync_period
      settings: SourceProductName=CASPER DSP Blockset
  fringe_theta_out : Outport  VectorParamsAs1DForOutWhenUnconnected=off
  wires:
  posedge1/1 -> Logical1/1, Logical3/2
  Logical1/1 -> Convert1/1
  FFT_Chnl_Cnt1/1 -> Relational1/1
  FFT_Length1/1 -> Relational1/2
  Convert1/1 -> FFT_Cycle_Cnt1/1
  Relational1/1 -> FFT_Cycle_Cnt1/2
  FFT_Cycle_Cnt1/1 -> Relational2/1
  Fringe_Rate_Reg1/1 -> Relational2/2
  Relational2/1 -> posedge1/1
  pulse_ext/1 -> Logical2/2
  Logical2/1 -> Delay1/1
  Delay1/1 -> Fringe_Theta_Cnt/1, fstop_mux/2
  Delay2/1 -> Logical3/1
  fstop_sel1/1 -> Relational_sel/1
  Relational_sel/1 -> fstop_mux/1
  Logical3/1 -> fstop_mux/3
  fstop_mux/1 -> Fringe_Theta_Cnt/3
  Fringe_Theta_Cnt/1 -> Delay3/1
  Delay3/1 -> Reinterpret/1
  en_theta_fs/1 -> pulse_ext/1
  theta_fs/1 -> Fringe_Theta_Cnt/2
  sync/1 -> Logical2/1, Delay2/1, Logical1/2, FFT_Chnl_Cnt1/1, Fringe_Rate_Reg1/2
  Reinterpret/1 -> fringe_theta_out/1
  fft_fs/1 -> Fringe_Rate_Reg1/1, Relational_sel/2

== system casper_library_delays/data_delay_gen ==
  sync_sgtemp : Inport
  delay_sgtemp : Inport  Port=2
  sync_out_sgtemp : Outport  VectorParamsAs1DForOutWhenUnconnected=off

== system casper_library_delays/delay_bram ==
  din : Inport
  constant : xbsIndex_r4/Constant  const=1  gui_display_data_type=Fixed-point  arith_type=Boolean  n_bits=16  bin_pt=14  preci_type=Single  exp_width=8  frac_width=24  explicit_period=on  period=1  equ=P=C  opselect=C  inp2=PCIN>>17  opr=+  inp1=P  carry=CIN  dbl_ovrd=off  block_type=constant
  counter : xbsIndex_r4/Counter  cnt_type=Count Limited  cnt_to=DelayLen - bram_latency - 1  operation=Up  start_count=0  cnt_by_val=1  arith_type=Unsigned  n_bits=2  bin_pt=0  load_pin=off  rst=off  en=off  explicit_period=on  period=1  use_behavioral_HDL=on  implementation=Fabric  use_rpm=off  dbl_ovrd=off  block_type=counter
  ram : xbsIndex_r4/Single Port RAM  depth=4  initVector=0  distributed_mem=Block RAM  write_mode=Read Before Write  rst=off  init_reg=0  en=off  optimize_latency=off  latency=bram_latency  optimize=Area  dbl_ovrd=off  simulation_type=fast_sim  block_type=spram
  dout : Outport  VectorParamsAs1DForOutWhenUnconnected=off
  wires:
  counter/1 -> ram/1
  din/1 -> ram/2
  constant/1 -> ram/3
  ram/1 -> dout/1

== system casper_library_delays/delay_bram_en_plus ==
  din : Inport
  en : Inport  Port=2
  Counter : xbsIndex_r4/Counter  cnt_type=Count Limited  cnt_to=DelayLen - 1  operation=Up  start_count=0  cnt_by_val=1  arith_type=Unsigned  n_bits=BitWidth  bin_pt=0  load_pin=off  rst=off  en=on  explicit_period=off  period=1  use_behavioral_HDL=off  implementation=Fabric  use_rpm=off  dbl_ovrd=off  block_type=counter
      settings: xl_area=[0, 0, 0, 0, 0, 0, 0]  block_version=9.1.01
  Delay : xbsIndex_r4/Delay  rst=off  infoeditControl=Selection of Reset will increase slice count due to use of real FFs and instead of SRLs  en=off  latency=bram_latency  reg_retiming=off  dbl_ovrd=off  block_type=delay
      settings: xl_area=[0, 0, 0, 0, 0, 0, 0]  block_version=9.1.01
  Single Port RAM : xbsIndex_r4/Single Port RAM  depth=2^BitWidth  initVector=0  distributed_mem=Block RAM  write_mode=Read Before Write  rst=off  init_reg=0  en=off  optimize_latency=off  latency=bram_latency  optimize=Area  dbl_ovrd=off  simulation_type=fast_sim  block_type=spram
      settings: xl_area=[0, 0, 0, 0, 0, 0, 0]  block_version=9.1.01
  dout : Outport  VectorParamsAs1DForOutWhenUnconnected=off
  valid : Outport  Port=2  VectorParamsAs1DForOutWhenUnconnected=off
  wires:
  Single Port RAM/1 -> dout/1
  Counter/1 -> Single Port RAM/1
  din/1 -> Single Port RAM/2
  en/1 -> Single Port RAM/3, Counter/1, Delay/1
  Delay/1 -> valid/1

== system casper_library_delays/delay_bram_prog ==
  din : Inport
  delay : Inport  Port=2
  AddSub : xbsIndex_r4/AddSub  mode=Subtraction  use_carryin=off  use_carryout=off  en=off  latency=2  precision=User Defined  arith_type=Unsigned  n_bits=MaxDelay  bin_pt=0  quantization=Truncate  overflow=Wrap  use_behavioral_HDL=on  hw_selection=Fabric  pipelined=off  use_rpm=on  dbl_ovrd=off  block_type=addsub
      settings: xl_area=[0, 0, 0, 0, 0, 0, 0]  block_version=9.1.01
  Constant1 : xbsIndex_r4/Constant  const=bram_latency + 1  gui_display_data_type=Fixed-point  arith_type=Unsigned  n_bits=MaxDelay  bin_pt=0  preci_type=Single  exp_width=8  frac_width=24  explicit_period=on  period=1  equ=P=C  opselect=C  inp2=PCIN>>17  opr=+  inp1=P  carry=CIN  dbl_ovrd=off  block_type=constant
      settings: block_version=9.1.01
  Constant2 : xbsIndex_r4/Constant  const=1  gui_display_data_type=Fixed-point  arith_type=Boolean  n_bits=1  bin_pt=0  preci_type=Single  exp_width=8  frac_width=24  explicit_period=on  period=1  equ=P=C  opselect=C  inp2=PCIN>>17  opr=+  inp1=P  carry=CIN  dbl_ovrd=off  block_type=constant
      settings: block_version=9.1.01
  Counter : xbsIndex_r4/Counter  cnt_type=Free Running  cnt_to=inf  operation=Up  start_count=0  cnt_by_val=1  arith_type=Unsigned  n_bits=MaxDelay  bin_pt=0  load_pin=off  rst=on  en=off  explicit_period=on  period=1  use_behavioral_HDL=off  implementation=Fabric  use_rpm=off  dbl_ovrd=off  block_type=counter
      settings: xl_area=[0, 0, 0, 0, 0, 0, 0]  block_version=9.1.01
  Relational : xbsIndex_r4/Relational  mode=a>=b  op_type=Bool  en=off  latency=0  dbl_ovrd=off  block_type=relational
      settings: xl_area=[0, 0, 0, 0, 0, 0, 0]  block_version=9.1.01
  Single Port RAM : xbsIndex_r4/Single Port RAM  depth=2^MaxDelay  initVector=0  distributed_mem=Block RAM  write_mode=Read Before Write  rst=off  init_reg=0  en=off  optimize_latency=off  latency=bram_latency  optimize=Area  dbl_ovrd=off  simulation_type=fast_sim  block_type=spram
      settings: xl_area=[0, 0, 0, 0, 0, 0, 0]  block_version=9.1.01
  dout : Outport  VectorParamsAs1DForOutWhenUnconnected=off
  wires:
  Constant1/1 -> AddSub/2
  AddSub/1 -> Relational/2
  delay/1 -> AddSub/1
  Relational/1 -> Counter/1
  Single Port RAM/1 -> dout/1
  Counter/1 -> Relational/1, Single Port RAM/1
  din/1 -> Single Port RAM/2
  Constant2/1 -> Single Port RAM/3

== system casper_library_delays/delay_bram_prog_dp ==

== system casper_library_delays/delay_complex ==
  In1 : Inport
  c_to_ri : casper_library_misc/c_to_ri  n_bits=18  bin_pt=17
      settings: SourceProductName=CASPER DSP Blockset
  delay1 : $bdroot/delay_bram  DelayLen=delay  bram_latency=bram_latency  use_dsp48=off  async=off
  delay2 : $bdroot/delay_bram  DelayLen=delay  bram_latency=bram_latency  use_dsp48=off  async=off
  ri_to_c : casper_library_misc/ri_to_c
      settings: SourceProductName=CASPER DSP Blockset
  Out1 : Outport  VectorParamsAs1DForOutWhenUnconnected=off
  wires:
  ri_to_c/1 -> Out1/1
  In1/1 -> c_to_ri/1
  delay2/1 -> ri_to_c/2
  c_to_ri/2 -> delay2/1
  delay1/1 -> ri_to_c/1
  c_to_ri/1 -> delay1/1

== system casper_library_delays/delay_slr ==

== system casper_library_delays/delay_srl ==

== system casper_library_delays/delay_tree ==
  in : Inport
  delay_c1_r1 : xbsIndex_r4/Delay  rst=off  infoeditControl=Selection of Reset will increase slice count due to use of real FFs and instead of SRLs  en=off  latency=1  reg_retiming=off  dbl_ovrd=off  block_type=delay
      settings: block_version=11.4
  delay_c2_r1 : xbsIndex_r4/Delay  rst=off  infoeditControl=Selection of Reset will increase slice count due to use of real FFs and instead of SRLs  en=off  latency=1  reg_retiming=off  dbl_ovrd=off  block_type=delay
      settings: block_version=11.4
  delay_c2_r2 : xbsIndex_r4/Delay  rst=off  infoeditControl=Selection of Reset will increase slice count due to use of real FFs and instead of SRLs  en=off  latency=1  reg_retiming=off  dbl_ovrd=off  block_type=delay
      settings: block_version=11.4
  out1 : Outport  VectorParamsAs1DForOutWhenUnconnected=off
  out2 : Outport  Port=2  VectorParamsAs1DForOutWhenUnconnected=off
  wires:
  in/1 -> delay_c1_r1/1
  delay_c1_r1/1 -> delay_c2_r1/1, delay_c2_r2/1
  delay_c2_r1/1 -> out1/1
  delay_c2_r2/1 -> out2/1

== system casper_library_delays/delay_wideband_prog ==
